simulink library "Linkage_Shock"  (R2025a)
settings: Solver=VariableStepAuto  StartTime=0.0  StopTime=10.0  RelTol=1e-3
undefined symbols (not defined in the file): bumpstop_len_shock, clr_conn_shock, clr_shock_bumpstop, clr_shock_cyl, clr_shock_piston, cyl_cap_len_shock, deadvol_len_shock_cyl, hp_spr_bot, hp_spr_top, low_lim_bumpstop, opc_conn_shock, opc_shock_bumpstop, opc_shock_cyl, opc_shock_piston, piston_len_shock, radius_shock_cyl, shock_cyl_mass, shock_pist_mass, size_conn_shock, up_lim_bumpstop, Vehicle, Visual, X, Y, Z
libraries: sm_lib x36, nesl_utility x9, fl_lib x3, Suspension_Utilities x3
(part 1 of 2)
Description:
  | Component of Simscape Vehicle Templates Library
  | 
  | Copyright 2018-2026 The MathWorks, Inc.
settings Model: Creator=smiller  LastModifiedBy=smiller
settings SolverCC: AlgebraicLoopSolver=TrustRegion
settings DataIOCC: ReturnWorkspaceOutputs=off
settings OptimizationCC: ReuseModelBlockBuffer=off
settings DebuggingCC: UnconnectedInputMsg=warning  UnconnectedOutputMsg=warning  UnconnectedLineMsg=warning  ArithmeticOperatorsInVariantConditions=warning
settings ModelReferenceCC: EnableRefExpFcnMdlSchedulingChecks=on
settings SFSimCC: CustomCodeUndefinedFunction=UseInterfaceOnly
settings RTWCC: GPUComputeCapability=3.5

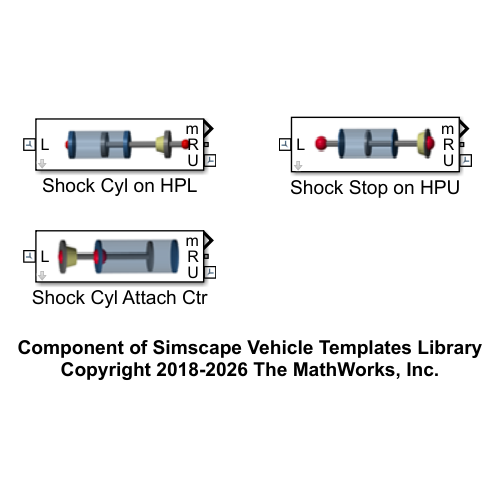
[thumbnail: Simulink's stored preview of the top-level diagram]
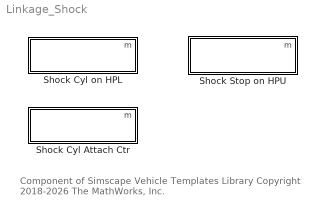
== system Linkage_Shock ==
  note: Component of Simscape Vehicle Templates Library
      | Copyright 2018-2026 The MathWorks, Inc.
  Shock Cyl Attach Ctr : Subsystem  mask(Shock Absorber Parts){shock_pist_mass=Vehicle.Chassis.SuspA1.AxleTA2PR.Shock.mPiston.Value, shock_cyl_mass=Vehicle.Chassis.SuspA1.AxleTA2PR.Shock.mCylinder.Value, hp_spr_top=Vehicle.Chassis.SuspA1.AxleTA2PR.Shock.sTop.Value, hp_spr_bot=Vehicle.Chassis.SuspA1.AxleTA2PR.Shock.sBottom.Value, up_lim_bumpstop=Vehicle.Chassis.SuspA1.AxleTA2PR.Endstop.xMax.Value, low_lim_bumpstop=Vehicle.Chassis.SuspA1.AxleTA2PR.Endstop.xMin.Value, clr_conn_shock=Visual.hp.clr, opc_conn_shock=Visual.hp.opc, size_conn_shock=Visual.hp.rad, clr_shock_cyl=Visual.clr.blue, opc_shock_cyl=Visual.part.opc, radius_shock_cyl=0.05, clr_shock_piston=Visual.clr.gray, opc_shock_piston=Visual.part.opc, clr_shock_bumpstop=Visual.clr.yellowpale, opc_shock_bumpstop=Visual.part.opc, deadvol_len_shock_cyl=Visual.Shock.dead_length, piston_len_shock=Visual.Shock.piston.len, cyl_cap_len_shock=Visual.Shock.cap.len, bumpstop_len_shock=Visual.Shock.bumpstop.len}
      mask prompts: shock_pist_mass "Piston Mass (kg)"; shock_cyl_mass "Cylinder Mass (kg)"; hp_spr_top "Spring Top [xyz] (m)"; hp_spr_bot "Spring Bottom [xyz] (m)"; up_lim_bumpstop "Upper Limit Bumpstop (m)"; low_lim_bumpstop "Lower Limit Bumpstop (m)"; deadvol_len_shock_cyl "Dead Volume Height (m)"; piston_len_shock "Piston Length (m)"; cyl_cap_len_shock "Cylinder Cap Length (m)"; bumpstop_len_shock "Bumpstop Length (m)"
      mask help: Models mechanical parts of shock absorber.
      mask init:
      | init_spr_len = norm(hp_spr_top-hp_spr_bot);
      | 
      | rod_length = init_spr_len+abs(up_lim_bumpstop)+piston_len_shock;
      | 
      | bumpstop_xc_rev = [0 0; 0.5 0; 0.7 1; 0 1].*[radius_shock_cyl bumpstop_len_shock];
      | 
      | cyl_wall_length = piston_len_shock+abs(low_lim_bumpstop)+abs(up_lim_bumpstop)+deadvol_len_shock_cyl;
      mask Help: web('sm_car_doc_susp_shock.html')
      mask TypeOptions shock_pist_mass: Piston/Rod/Mass
      mask TypeOptions shock_cyl_mass: Cylinder/Wall/Mass
      mask TypeOptions clr_conn_shock:
      | Vis
      | Spring
      | LA/GraphicDiffuseColor | Vis
      | Spring
      | HP/GraphicDiffuseColor
      mask TypeOptions opc_conn_shock:
      | Vis
      | Spring
      | LA/GraphicOpacity | Vis
      | Spring
      | HP/GraphicOpacity
      mask TypeOptions clr_shock_cyl: Cylinder/Cap Bottom/GraphicDiffuseColor | Cylinder/Cap Top/GraphicDiffuseColor | Cylinder/Wall/GraphicDiffuseColor
      mask TypeOptions clr_shock_piston: Piston/Cap/GraphicDiffuseColor | Piston/Piston/GraphicDiffuseColor | Piston/Rod/GraphicDiffuseColor
      mask TypeOptions opc_shock_piston: Piston/Cap/GraphicOpacity | Piston/Piston/GraphicOpacity | Piston/Rod/GraphicOpacity
      mask TypeOptions clr_shock_bumpstop: Piston/Bumpstop/GraphicDiffuseColor
      mask TypeOptions opc_shock_bumpstop: Piston/Bumpstop/GraphicOpacity
      mask DialogControl cont_shock Prompt: Shock
      mask DialogControl cont_vis_shock Prompt: Visualization
      mask DialogControl text_clr_shock Prompt: Color  [RGB]
      mask DialogControl text_opc_shock Prompt: Opac. (0-1)
      mask DialogControl text_size_shock Prompt: Size (m)
      mask DialogControl text_conn_shock Prompt: Connections
      mask DialogControl text_shock_cyl Prompt: Cylinder
      mask DialogControl text_shock_piston Prompt: Piston
      mask DialogControl text_piston_radius Prompt: <cylinder radius>
      mask DialogControl text_shock_bumpstop Prompt: Bumpstop
      mask DialogControl text_bumpstop_radius Prompt: <cylinder radius>
      mask Display: image('sm_car_vehicle_linkage_shock_hpc_IMAGE.png');
  Shock Cyl on HPL : Subsystem  mask{shock_pist_mass=shock_pist_mass, shock_cyl_mass=shock_cyl_mass, hp_spr_top=hp_spr_top, hp_spr_bot=hp_spr_bot, up_lim_bumpstop=up_lim_bumpstop, low_lim_bumpstop=low_lim_bumpstop, clr_conn_shock=clr_conn_shock, opc_conn_shock=opc_conn_shock, size_conn_shock=size_conn_shock, clr_shock_cyl=clr_shock_cyl, opc_shock_cyl=opc_shock_cyl, radius_shock_cyl=radius_shock_cyl, clr_shock_piston=clr_shock_piston, opc_shock_piston=opc_shock_piston, clr_shock_bumpstop=clr_shock_bumpstop, opc_shock_bumpstop=opc_shock_bumpstop, deadvol_len_shock_cyl=deadvol_len_shock_cyl, piston_len_shock=piston_len_shock, cyl_cap_len_shock=cyl_cap_len_shock, bumpstop_len_shock=bumpstop_len_shock}
      mask prompts: shock_pist_mass "Piston Mass (kg)"; shock_cyl_mass "Cylinder Mass (kg)"; hp_spr_top "Shock Top [xyz] (m)"; hp_spr_bot "Shock Bottom [xyz] (m)"; up_lim_bumpstop "Upper Limit Bumpstop (m)"; low_lim_bumpstop "Lower Limit Bumpstop (m)"; deadvol_len_shock_cyl "Dead Volume Height (m)"; piston_len_shock "Piston Length (m)"; cyl_cap_len_shock "Cylinder Cap Length (m)"; bumpstop_len_shock "Bumpstop Length (m)"
      mask init:
      | init_spr_len = norm(hp_spr_top-hp_spr_bot);
      | 
      | rod_length = init_spr_len-deadvol_len_shock_cyl-cyl_cap_len_shock-abs(low_lim_bumpstop);
      | 
      | bumpstop_xc_rev = [0 0; 0.7 0; 0.9 1; 0 1].*[radius_shock_cyl bumpstop_len_shock];
      | 
      | cyl_wall_length = piston_len_shock+abs(low_lim_bumpstop)+abs(up_lim_bumpstop)+deadvol_len_shock_cyl;
      mask Help: web('sm_car_doc_susp_shock.html')
      mask TypeOptions shock_pist_mass: Piston/Rod/Mass
      mask TypeOptions shock_cyl_mass: Cylinder/Wall/Mass
      mask TypeOptions clr_conn_shock:
      | Vis
      | HP L/GraphicDiffuseColor | Vis
      | HP U/GraphicDiffuseColor
      mask TypeOptions opc_conn_shock:
      | Vis
      | HP L/GraphicOpacity | Vis
      | HP U/GraphicOpacity
      mask TypeOptions clr_shock_cyl: Cylinder/Cap Bottom/GraphicDiffuseColor | Cylinder/Cap Top/GraphicDiffuseColor | Cylinder/Wall/GraphicDiffuseColor
      mask TypeOptions clr_shock_piston: Piston/Cap/GraphicDiffuseColor | Piston/Piston/GraphicDiffuseColor | Piston/Rod/GraphicDiffuseColor
      mask TypeOptions opc_shock_piston: Piston/Cap/GraphicOpacity | Piston/Piston/GraphicOpacity | Piston/Rod/GraphicOpacity
      mask TypeOptions clr_shock_bumpstop: Piston/Bumpstop/GraphicDiffuseColor
      mask TypeOptions opc_shock_bumpstop: Piston/Bumpstop/GraphicOpacity
      mask DialogControl cont_shock Prompt: Shock
      mask DialogControl cont_vis_shock Prompt: Visualization
      mask DialogControl text_blank_shock Prompt: (Add text here)
      mask DialogControl text_clr_shock Prompt: Color  [RGB]
      mask DialogControl text_opc_shock Prompt: Opac. (0-1)
      mask DialogControl text_size_shock Prompt: Size (m)
      mask DialogControl text_conn_shock Prompt: Connections
      mask DialogControl text_shock_cyl Prompt: Cylinder
      mask DialogControl text_shock_piston Prompt: Piston
      mask DialogControl text_piston_radius Prompt: <cylinder radius>
      mask DialogControl text_shock_bumpstop Prompt: Bumpstop
      mask DialogControl text_bumpstop_radius Prompt: <cylinder radius>
      mask Display: image('sm_car_vehicle_linkage_shock_IMAGE.png');
  Shock Stop on HPU : Subsystem  mask{shock_pist_mass=shock_pist_mass, shock_cyl_mass=shock_cyl_mass, hp_spr_top=hp_spr_top, hp_spr_bot=hp_spr_bot, up_lim_bumpstop=up_lim_bumpstop, low_lim_bumpstop=low_lim_bumpstop, clr_conn_shock=clr_conn_shock, opc_conn_shock=opc_conn_shock, size_conn_shock=size_conn_shock, clr_shock_cyl=clr_shock_cyl, opc_shock_cyl=opc_shock_cyl, radius_shock_cyl=radius_shock_cyl, clr_shock_piston=clr_shock_piston, opc_shock_piston=opc_shock_piston, clr_shock_bumpstop=clr_shock_bumpstop, opc_shock_bumpstop=opc_shock_bumpstop, deadvol_len_shock_cyl=deadvol_len_shock_cyl, piston_len_shock=piston_len_shock, cyl_cap_len_shock=cyl_cap_len_shock, bumpstop_len_shock=bumpstop_len_shock}
      mask prompts: shock_pist_mass "Piston Mass (kg)"; shock_cyl_mass "Cylinder Mass (kg)"; hp_spr_top "Shock Top [xyz] (m)"; hp_spr_bot "Shock Bottom [xyz] (m)"; up_lim_bumpstop "Upper Limit Bumpstop (m)"; low_lim_bumpstop "Lower Limit Bumpstop (m)"; deadvol_len_shock_cyl "Dead Volume Height (m)"; piston_len_shock "Piston Length (m)"; cyl_cap_len_shock "Cylinder Cap Length (m)"; bumpstop_len_shock "Bumpstop Length (m)"
      mask init:
      | init_spr_len = norm(hp_spr_top-hp_spr_bot);
      | 
      | rod_length_upper = ...
      | cyl_cap_len_shock + bumpstop_len_shock + abs(low_lim_bumpstop) + ...
      | cyl_cap_len_shock + abs(up_lim_bumpstop) + piston_len_shock;
      | 
      | rod_length_lower = init_spr_len - rod_length_upper - deadvol_len_shock_cyl - cyl_cap_len_shock - abs(low_lim_bumpstop);
      | 
      | bumpstop_xc_rev = [0 0; 0.7 0; 0.9 1; 0 1].*[radius_shock_cyl bumpstop_len_shock];
      | 
      | cyl_wall_length = piston_len_shock+abs(low_lim_bumpstop)+abs(up_lim_bumpstop)+deadvol_len_shock_cyl;
      mask Help: web('sm_car_doc_susp_shock.html')
      mask TypeOptions shock_pist_mass: Piston/Rod/Mass
      mask TypeOptions shock_cyl_mass: Cylinder/Wall/Mass
      mask TypeOptions clr_conn_shock:
      | Vis
      | HP L/GraphicDiffuseColor | Vis
      | HP U/GraphicDiffuseColor
      mask TypeOptions opc_conn_shock:
      | Vis
      | HP L/GraphicOpacity | Vis
      | HP U/GraphicOpacity
      mask TypeOptions clr_shock_cyl: Cylinder/Cap Bottom/GraphicDiffuseColor | Cylinder/Cap Top/GraphicDiffuseColor | Cylinder/Wall/GraphicDiffuseColor
      mask TypeOptions clr_shock_piston: Piston/Cap/GraphicDiffuseColor | Piston/Piston/GraphicDiffuseColor | Piston/Rod/GraphicDiffuseColor
      mask TypeOptions opc_shock_piston: Piston/Cap/GraphicOpacity | Piston/Piston/GraphicOpacity | Piston/Rod/GraphicOpacity
      mask TypeOptions clr_shock_bumpstop: Piston/Bumpstop/GraphicDiffuseColor
      mask TypeOptions opc_shock_bumpstop: Piston/Bumpstop/GraphicOpacity
      mask DialogControl cont_shock Prompt: Shock
      mask DialogControl cont_vis_shock Prompt: Visualization
      mask DialogControl text_blank_shock Prompt: (Add text here)
      mask DialogControl text_clr_shock Prompt: Color  [RGB]
      mask DialogControl text_opc_shock Prompt: Opac. (0-1)
      mask DialogControl text_size_shock Prompt: Size (m)
      mask DialogControl text_conn_shock Prompt: Connections
      mask DialogControl text_shock_cyl Prompt: Cylinder
      mask DialogControl text_shock_piston Prompt: Piston
      mask DialogControl text_piston_radius Prompt: <cylinder radius>
      mask DialogControl text_shock_bumpstop Prompt: Bumpstop
      mask DialogControl text_bumpstop_radius Prompt: <cylinder radius>
      mask Display: image('sm_car_vehicle_linkage_shock_hpu_IMAGE.png');

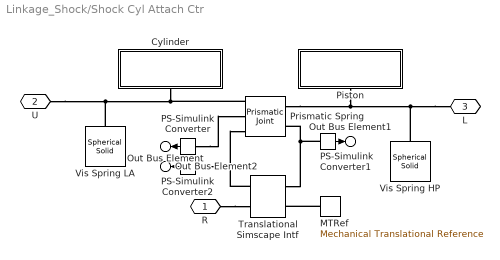
== system Linkage_Shock/Shock Cyl Attach Ctr ==
  Cylinder : Subsystem
  MTRef : fl_lib/Mechanical/Translational Elements/Mechanical Translational Reference
  PS-Simulink Converter : nesl_utility/PS-Simulink Converter  PhysicalDomain=network_engine_domain  SubClassName=ps_output  LeftPortType=input  RightPortType=output  PseudoPeriodic=off  Frequencies=[]  VectorFormat=1-D array  Unit=1  AffineConversion=off
  PS-Simulink Converter1 : nesl_utility/PS-Simulink Converter  PhysicalDomain=network_engine_domain  SubClassName=ps_output  LeftPortType=input  RightPortType=output  PseudoPeriodic=off  Frequencies=[]  VectorFormat=1-D array  Unit=1  AffineConversion=off
  PS-Simulink Converter2 : nesl_utility/PS-Simulink Converter  PhysicalDomain=network_engine_domain  SubClassName=ps_output  LeftPortType=input  RightPortType=output  PseudoPeriodic=off  Frequencies=[]  VectorFormat=1-D array  Unit=1  AffineConversion=off
  Piston : Subsystem
  Prismatic Spring : sm_lib/Joints/Prismatic Joint  JointMode=Normal  CompositeWrenchDir=FollowerOnBase  CompositeWrenchFrame=BaseFrame  SenseConstraintForce=off  SenseConstraintTorque=off  SenseTotalForce=off  SenseTotalTorque=off  PositionTargetSpecify=on  PositionTargetPriority=Low  PositionTargetValue=init_spr_len  PositionTargetValueUnits=m  VelocityTargetSpecify=off  VelocityTargetPriority=High  VelocityTargetValue=0  VelocityTargetValueUnits=m/s  EquilibriumPosition=0  EquilibriumPositionUnits=m  SpringStiffness=0  SpringStiffnessUnits=N/m  DampingCoefficient=0.01  DampingCoefficientUnits=N/(m/s)  LowerLimitSpecify=off  LowerLimitBound=-1  LowerLimitBoundUnits=m  LowerLimitStiffness=1e6  LowerLimitStiffnessUnits=N/m  LowerLimitDamping=1e3  LowerLimitDampingUnits=N/(m/s)  LowerLimitTransitionRegionWidth=1e-4  LowerLimitTransitionRegionWidthUnits=m  UpperLimitSpecify=off  UpperLimitBound=1  UpperLimitBoundUnits=m  UpperLimitStiffness=1e6  UpperLimitStiffnessUnits=N/m  UpperLimitDamping=1e3  UpperLimitDampingUnits=N/(m/s)  UpperLimitTransitionRegionWidth=1e-4  UpperLimitTransitionRegionWidthUnits=m  TorqueActuationMode=InputTorque  MotionActuationMode=ComputedMotion  SensePosition=on  SenseVelocity=on  SenseAcceleration=off  SenseTorqueForce=off  SenseLowerLimitTorqueForce=off  SenseUpperLimitTorqueForce=off
  Translational Simscape Intf : Suspension_Utilities/Translational Simscape Intf  SystemSampleTime=-1  VariantActivationTime=update diagram  EmptyChoice=off  PassThrough=off  PassThroughVariantControl=(default)  EmptyChoiceVariantControl=(default)  AllowFlexibleInterface=on  Latency=0  AutoFrameSizeCalculation=off
  Vis Spring HP : sm_lib/Body Elements/Spherical Solid  SphereRadius=size_conn_shock  SphereRadiusUnits=m  ExportEntireGeometry=off  InertiaType=PointMass  BasedOnType=Density  Density=0  DensityUnits=kg/m^3  Mass=0  MassUnits=kg  CenterOfMass=[0 0 0]  CenterOfMassUnits=m  MomentsOfInertia=[1 1 1]  MomentsOfInertiaUnits=kg*m^2  ProductsOfInertia=[0 0 0]  ProductsOfInertiaUnits=kg*m^2  GraphicType=FromGeometry  MarkerShape=Sphere  MarkerSize=10  GraphicVisPropType=SimpleVisualProperties  GraphicDiffuseColor=clr_conn_shock  GraphicOpacity=opc_conn_shock  GraphicSpecularColor=[0.5 0.5 0.5 1.0]  GraphicAmbientColor=[0.15 0.15 0.15 1.0]  GraphicEmissiveColor=[0.0 0.0 0.0 1.0]  GraphicShininess=75  DoExposeReferenceFrame=on  SerializedFrames=<Frames/>
  Vis Spring LA : sm_lib/Body Elements/Spherical Solid  SphereRadius=size_conn_shock  SphereRadiusUnits=m  ExportEntireGeometry=off  InertiaType=PointMass  BasedOnType=Density  Density=0  DensityUnits=kg/m^3  Mass=0  MassUnits=kg  CenterOfMass=[0 0 0]  CenterOfMassUnits=m  MomentsOfInertia=[1 1 1]  MomentsOfInertiaUnits=kg*m^2  ProductsOfInertia=[0 0 0]  ProductsOfInertiaUnits=kg*m^2  GraphicType=FromGeometry  MarkerShape=Sphere  MarkerSize=10  GraphicVisPropType=SimpleVisualProperties  GraphicDiffuseColor=clr_conn_shock  GraphicOpacity=opc_conn_shock  GraphicSpecularColor=[0.5 0.5 0.5 1.0]  GraphicAmbientColor=[0.15 0.15 0.15 1.0]  GraphicEmissiveColor=[0.0 0.0 0.0 1.0]  GraphicShininess=75  DoExposeReferenceFrame=on  SerializedFrames=<Frames/>
  R : PMIOPort  Side=Right
  U : PMIOPort  Port=2  Side=Right
  L : PMIOPort  Port=3  Side=Left
  Out Bus Element : Outport  VectorParamsAs1DForOutWhenUnconnected=off  PortName=m  Element=x
  Out Bus Element1 : Outport  VectorParamsAs1DForOutWhenUnconnected=off  PortName=m  Element=f
  Out Bus Element2 : Outport  VectorParamsAs1DForOutWhenUnconnected=off  PortName=m  Element=v
  wires:
  PS-Simulink Converter/1 -> Out Bus Element/1
  PS-Simulink Converter1/1 -> Out Bus Element1/1
  PS-Simulink Converter2/1 -> Out Bus Element2/1
  connections:
  R/RConn1 -- Translational Simscape Intf/RConn2
  MTRef/LConn1 -- Translational Simscape Intf/LConn2
  L/RConn1 -- Prismatic Spring/LConn1 -- Piston/RConn1 -- Vis Spring HP/RConn1
  Cylinder/LConn1 -- U/RConn1 -- Vis Spring LA/RConn1 -- Prismatic Spring/RConn1
  Translational Simscape Intf/RConn1 -- PS-Simulink Converter2/LConn1 -- Prismatic Spring/RConn3
  Translational Simscape Intf/LConn1 -- PS-Simulink Converter1/LConn1 -- Prismatic Spring/LConn2
  PS-Simulink Converter/LConn1 -- Prismatic Spring/RConn2

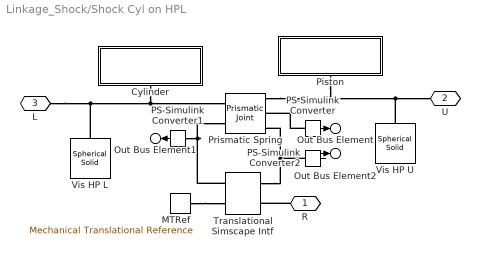
== system Linkage_Shock/Shock Cyl on HPL ==
  Cylinder : Subsystem
  MTRef : fl_lib/Mechanical/Translational Elements/Mechanical Translational Reference
  PS-Simulink Converter : nesl_utility/PS-Simulink Converter  PhysicalDomain=network_engine_domain  SubClassName=ps_output  LeftPortType=input  RightPortType=output  PseudoPeriodic=off  Frequencies=[]  VectorFormat=1-D array  Unit=m  AffineConversion=off
  PS-Simulink Converter1 : nesl_utility/PS-Simulink Converter  PhysicalDomain=network_engine_domain  SubClassName=ps_output  LeftPortType=input  RightPortType=output  PseudoPeriodic=off  Frequencies=[]  VectorFormat=1-D array  Unit=N  AffineConversion=off
  PS-Simulink Converter2 : nesl_utility/PS-Simulink Converter  PhysicalDomain=network_engine_domain  SubClassName=ps_output  LeftPortType=input  RightPortType=output  PseudoPeriodic=off  Frequencies=[]  VectorFormat=1-D array  Unit=m/s  AffineConversion=off
  Piston : Subsystem
  Prismatic Spring : sm_lib/Joints/Prismatic Joint  JointMode=Normal  CompositeWrenchDir=FollowerOnBase  CompositeWrenchFrame=BaseFrame  SenseConstraintForce=off  SenseConstraintTorque=off  SenseTotalForce=off  SenseTotalTorque=off  PositionTargetSpecify=on  PositionTargetPriority=High  PositionTargetValue=init_spr_len  PositionTargetValueUnits=m  VelocityTargetSpecify=off  VelocityTargetPriority=High  VelocityTargetValue=0  VelocityTargetValueUnits=m/s  EquilibriumPosition=0  EquilibriumPositionUnits=m  SpringStiffness=0  SpringStiffnessUnits=N/m  DampingCoefficient=0.01  DampingCoefficientUnits=N/(m/s)  LowerLimitSpecify=off  LowerLimitBound=-1  LowerLimitBoundUnits=m  LowerLimitStiffness=1e6  LowerLimitStiffnessUnits=N/m  LowerLimitDamping=1e3  LowerLimitDampingUnits=N/(m/s)  LowerLimitTransitionRegionWidth=1e-4  LowerLimitTransitionRegionWidthUnits=m  UpperLimitSpecify=off  UpperLimitBound=1  UpperLimitBoundUnits=m  UpperLimitStiffness=1e6  UpperLimitStiffnessUnits=N/m  UpperLimitDamping=1e3  UpperLimitDampingUnits=N/(m/s)  UpperLimitTransitionRegionWidth=1e-4  UpperLimitTransitionRegionWidthUnits=m  TorqueActuationMode=InputTorque  MotionActuationMode=ComputedMotion  SensePosition=on  SenseVelocity=on  SenseAcceleration=off  SenseTorqueForce=off  SenseLowerLimitTorqueForce=off  SenseUpperLimitTorqueForce=off
  Translational Simscape Intf : Suspension_Utilities/Translational Simscape Intf  SystemSampleTime=-1  VariantActivationTime=update diagram  EmptyChoice=off  PassThrough=off  PassThroughVariantControl=(default)  EmptyChoiceVariantControl=(default)  AllowFlexibleInterface=on  Latency=0  AutoFrameSizeCalculation=off
  Vis HP L : sm_lib/Body Elements/Spherical Solid  SphereRadius=size_conn_shock  SphereRadiusUnits=m  ExportEntireGeometry=off  InertiaType=PointMass  BasedOnType=Density  Density=0  DensityUnits=kg/m^3  Mass=0  MassUnits=kg  CenterOfMass=[0 0 0]  CenterOfMassUnits=m  MomentsOfInertia=[1 1 1]  MomentsOfInertiaUnits=kg*m^2  ProductsOfInertia=[0 0 0]  ProductsOfInertiaUnits=kg*m^2  GraphicType=FromGeometry  MarkerShape=Sphere  MarkerSize=10  GraphicVisPropType=SimpleVisualProperties  GraphicDiffuseColor=clr_conn_shock  GraphicOpacity=opc_conn_shock  GraphicSpecularColor=[0.5 0.5 0.5 1.0]  GraphicAmbientColor=[0.15 0.15 0.15 1.0]  GraphicEmissiveColor=[0.0 0.0 0.0 1.0]  GraphicShininess=75  DoExposeReferenceFrame=on  SerializedFrames=<Frames/>
  Vis HP U : sm_lib/Body Elements/Spherical Solid  SphereRadius=size_conn_shock  SphereRadiusUnits=m  ExportEntireGeometry=off  InertiaType=PointMass  BasedOnType=Density  Density=0  DensityUnits=kg/m^3  Mass=0  MassUnits=kg  CenterOfMass=[0 0 0]  CenterOfMassUnits=m  MomentsOfInertia=[1 1 1]  MomentsOfInertiaUnits=kg*m^2  ProductsOfInertia=[0 0 0]  ProductsOfInertiaUnits=kg*m^2  GraphicType=FromGeometry  MarkerShape=Sphere  MarkerSize=10  GraphicVisPropType=SimpleVisualProperties  GraphicDiffuseColor=clr_conn_shock  GraphicOpacity=opc_conn_shock  GraphicSpecularColor=[0.5 0.5 0.5 1.0]  GraphicAmbientColor=[0.15 0.15 0.15 1.0]  GraphicEmissiveColor=[0.0 0.0 0.0 1.0]  GraphicShininess=75  DoExposeReferenceFrame=on  SerializedFrames=<Frames/>
  R : PMIOPort  Side=Right
  U : PMIOPort  Port=2  Side=Right
  L : PMIOPort  Port=3  Side=Left
  Out Bus Element : Outport  VectorParamsAs1DForOutWhenUnconnected=off  PortName=m  Element=x
  Out Bus Element1 : Outport  VectorParamsAs1DForOutWhenUnconnected=off  PortName=m  Element=f
  Out Bus Element2 : Outport  VectorParamsAs1DForOutWhenUnconnected=off  PortName=m  Element=v
  wires:
  PS-Simulink Converter/1 -> Out Bus Element/1
  PS-Simulink Converter1/1 -> Out Bus Element1/1
  PS-Simulink Converter2/1 -> Out Bus Element2/1
  connections:
  Translational Simscape Intf/LConn1 -- PS-Simulink Converter1/LConn1 -- Prismatic Spring/LConn2
  Translational Simscape Intf/RConn1 -- PS-Simulink Converter2/LConn1 -- Prismatic Spring/RConn3
  Vis HP L/RConn1 -- Cylinder/LConn1 -- Prismatic Spring/LConn1 -- L/RConn1
  Vis HP U/RConn1 -- Piston/RConn1 -- Prismatic Spring/RConn1 -- U/RConn1
  MTRef/LConn1 -- Translational Simscape Intf/LConn2
  R/RConn1 -- Translational Simscape Intf/RConn2
  PS-Simulink Converter/LConn1 -- Prismatic Spring/RConn2

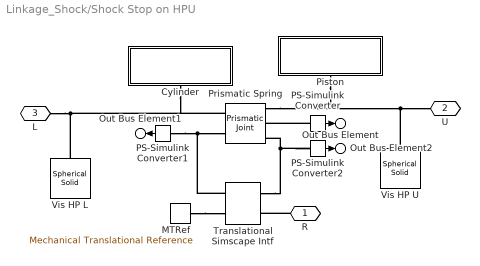
== system Linkage_Shock/Shock Stop on HPU ==
  Cylinder : Subsystem
  MTRef : fl_lib/Mechanical/Translational Elements/Mechanical Translational Reference
  PS-Simulink Converter : nesl_utility/PS-Simulink Converter  PhysicalDomain=network_engine_domain  SubClassName=ps_output  LeftPortType=input  RightPortType=output  PseudoPeriodic=off  Frequencies=[]  VectorFormat=1-D array  Unit=m  AffineConversion=off
  PS-Simulink Converter1 : nesl_utility/PS-Simulink Converter  PhysicalDomain=network_engine_domain  SubClassName=ps_output  LeftPortType=input  RightPortType=output  PseudoPeriodic=off  Frequencies=[]  VectorFormat=1-D array  Unit=N  AffineConversion=off
  PS-Simulink Converter2 : nesl_utility/PS-Simulink Converter  PhysicalDomain=network_engine_domain  SubClassName=ps_output  LeftPortType=input  RightPortType=output  PseudoPeriodic=off  Frequencies=[]  VectorFormat=1-D array  Unit=m/s  AffineConversion=off
  Piston : Subsystem
  Prismatic Spring : sm_lib/Joints/Prismatic Joint  JointMode=Normal  CompositeWrenchDir=FollowerOnBase  CompositeWrenchFrame=BaseFrame  SenseConstraintForce=off  SenseConstraintTorque=off  SenseTotalForce=off  SenseTotalTorque=off  PositionTargetSpecify=on  PositionTargetPriority=High  PositionTargetValue=init_spr_len  PositionTargetValueUnits=m  VelocityTargetSpecify=off  VelocityTargetPriority=High  VelocityTargetValue=0  VelocityTargetValueUnits=m/s  EquilibriumPosition=0  EquilibriumPositionUnits=m  SpringStiffness=0  SpringStiffnessUnits=N/m  DampingCoefficient=0  DampingCoefficientUnits=N/(m/s)  LowerLimitSpecify=off  LowerLimitBound=-1  LowerLimitBoundUnits=m  LowerLimitStiffness=1e6  LowerLimitStiffnessUnits=N/m  LowerLimitDamping=1e3  LowerLimitDampingUnits=N/(m/s)  LowerLimitTransitionRegionWidth=1e-4  LowerLimitTransitionRegionWidthUnits=m  UpperLimitSpecify=off  UpperLimitBound=1  UpperLimitBoundUnits=m  UpperLimitStiffness=1e6  UpperLimitStiffnessUnits=N/m  UpperLimitDamping=1e3  UpperLimitDampingUnits=N/(m/s)  UpperLimitTransitionRegionWidth=1e-4  UpperLimitTransitionRegionWidthUnits=m  TorqueActuationMode=InputTorque  MotionActuationMode=ComputedMotion  SensePosition=on  SenseVelocity=on  SenseAcceleration=off  SenseTorqueForce=off  SenseLowerLimitTorqueForce=off  SenseUpperLimitTorqueForce=off
  Translational Simscape Intf : Suspension_Utilities/Translational Simscape Intf  SystemSampleTime=-1  VariantActivationTime=update diagram  EmptyChoice=off  PassThrough=off  PassThroughVariantControl=(default)  EmptyChoiceVariantControl=(default)  AllowFlexibleInterface=on  Latency=0  AutoFrameSizeCalculation=off
  Vis HP L : sm_lib/Body Elements/Spherical Solid  SphereRadius=size_conn_shock  SphereRadiusUnits=m  ExportEntireGeometry=off  InertiaType=PointMass  BasedOnType=Density  Density=0  DensityUnits=kg/m^3  Mass=0  MassUnits=kg  CenterOfMass=[0 0 0]  CenterOfMassUnits=m  MomentsOfInertia=[1 1 1]  MomentsOfInertiaUnits=kg*m^2  ProductsOfInertia=[0 0 0]  ProductsOfInertiaUnits=kg*m^2  GraphicType=FromGeometry  MarkerShape=Sphere  MarkerSize=10  GraphicVisPropType=SimpleVisualProperties  GraphicDiffuseColor=clr_conn_shock  GraphicOpacity=opc_conn_shock  GraphicSpecularColor=[0.5 0.5 0.5 1.0]  GraphicAmbientColor=[0.15 0.15 0.15 1.0]  GraphicEmissiveColor=[0.0 0.0 0.0 1.0]  GraphicShininess=75  DoExposeReferenceFrame=on  SerializedFrames=<Frames/>
  Vis HP U : sm_lib/Body Elements/Spherical Solid  SphereRadius=size_conn_shock  SphereRadiusUnits=m  ExportEntireGeometry=off  InertiaType=PointMass  BasedOnType=Density  Density=0  DensityUnits=kg/m^3  Mass=0  MassUnits=kg  CenterOfMass=[0 0 0]  CenterOfMassUnits=m  MomentsOfInertia=[1 1 1]  MomentsOfInertiaUnits=kg*m^2  ProductsOfInertia=[0 0 0]  ProductsOfInertiaUnits=kg*m^2  GraphicType=FromGeometry  MarkerShape=Sphere  MarkerSize=10  GraphicVisPropType=SimpleVisualProperties  GraphicDiffuseColor=clr_conn_shock  GraphicOpacity=opc_conn_shock  GraphicSpecularColor=[0.5 0.5 0.5 1.0]  GraphicAmbientColor=[0.15 0.15 0.15 1.0]  GraphicEmissiveColor=[0.0 0.0 0.0 1.0]  GraphicShininess=75  DoExposeReferenceFrame=on  SerializedFrames=<Frames/>
  R : PMIOPort  Side=Right
  U : PMIOPort  Port=2  Side=Right
  L : PMIOPort  Port=3  Side=Left
  Out Bus Element : Outport  VectorParamsAs1DForOutWhenUnconnected=off  PortName=m  Element=x
  Out Bus Element1 : Outport  VectorParamsAs1DForOutWhenUnconnected=off  PortName=m  Element=f
  Out Bus Element2 : Outport  VectorParamsAs1DForOutWhenUnconnected=off  PortName=m  Element=v
  wires:
  PS-Simulink Converter/1 -> Out Bus Element/1
  PS-Simulink Converter1/1 -> Out Bus Element1/1
  PS-Simulink Converter2/1 -> Out Bus Element2/1
  connections:
  R/RConn1 -- Translational Simscape Intf/RConn2
  MTRef/LConn1 -- Translational Simscape Intf/LConn2
  Piston/RConn1 -- Prismatic Spring/RConn1 -- Vis HP U/RConn1 -- U/RConn1
  Translational Simscape Intf/RConn1 -- PS-Simulink Converter2/LConn1 -- Prismatic Spring/RConn3
  Translational Simscape Intf/LConn1 -- PS-Simulink Converter1/LConn1 -- Prismatic Spring/LConn2
  L/RConn1 -- Prismatic Spring/LConn1 -- Cylinder/LConn1 -- Vis HP L/RConn1
  PS-Simulink Converter/LConn1 -- Prismatic Spring/RConn2

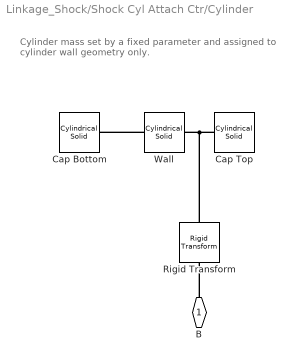
== system Linkage_Shock/Shock Cyl Attach Ctr/Cylinder ==
  note: Cylinder mass set by a fixed parameter
      | and assigned to cylinder wall geometry only.
  Cap Bottom : sm_lib/Body Elements/Cylindrical Solid  CylinderRadius=radius_shock_cyl  CylinderRadiusUnits=m  CylinderLength=cyl_cap_len_shock  CylinderLengthUnits=m  ExportEntireGeometry=off  InertiaType=CalculateFromGeometry  BasedOnType=Density  Density=0  DensityUnits=kg/m^3  Mass=1  MassUnits=kg  CenterOfMass=[0 0 0]  CenterOfMassUnits=m  MomentsOfInertia=[1 1 1]  MomentsOfInertiaUnits=kg*m^2  ProductsOfInertia=[0 0 0]  ProductsOfInertiaUnits=kg*m^2  GraphicType=FromGeometry  MarkerShape=Sphere  MarkerSize=10  GraphicVisPropType=SimpleVisualProperties  GraphicDiffuseColor=clr_shock_cyl  GraphicOpacity=opc_shock_cyl  GraphicSpecularColor=[0.5 0.5 0.5 1.0]  GraphicAmbientColor=[0.15 0.15 0.15 1.0]  GraphicEmissiveColor=[0.0 0.0 0.0 1.0]  GraphicShininess=75  DoExposeReferenceFrame=off  SerializedFrames=<Frames><Frame><Id>Frame1</Id><Value><Name>F</Name><Origin><Source>GeometricFeature</Source><FeatureName>top surface</FeatureName></Origin><PrimaryAxis><DefinedDirection>+Z</DefinedDirection><Source>ReferenceFrame</Source><SourceDirection>+Z</SourceDirection><FeatureName></FeatureName></PrimaryAxis><SecondaryAxis><DefinedDirection>+X</DefinedDirection><Source>ReferenceFrame</Source><SourceDirection>+X</SourceDirection><FeatureName></FeatureName></SecondaryAxis></Value></Frame><Frame><Id>Frame2</Id><Value><Name>B</Name><Origin><Source>GeometricFeature</Source><FeatureName>bottom surface</FeatureName></Origin><PrimaryAxis><DefinedDirection>+Z</DefinedDirection><Source>ReferenceFrame</Source><SourceDirection>+Z</SourceDirection><FeatureName></FeatureName></PrimaryAxis><SecondaryAxis><DefinedDirection>+X</DefinedDirection><Source>ReferenceFrame</Source><SourceDirection>+X</SourceDirection><FeatureName></FeatureName></SecondaryAxis></Value></Frame></Frames>
  Cap Top : sm_lib/Body Elements/Cylindrical Solid  CylinderRadius=radius_shock_cyl  CylinderRadiusUnits=m  CylinderLength=cyl_cap_len_shock  CylinderLengthUnits=m  ExportEntireGeometry=off  InertiaType=CalculateFromGeometry  BasedOnType=Density  Density=0  DensityUnits=kg/m^3  Mass=1  MassUnits=kg  CenterOfMass=[0 0 0]  CenterOfMassUnits=m  MomentsOfInertia=[1 1 1]  MomentsOfInertiaUnits=kg*m^2  ProductsOfInertia=[0 0 0]  ProductsOfInertiaUnits=kg*m^2  GraphicType=FromGeometry  MarkerShape=Sphere  MarkerSize=10  GraphicVisPropType=SimpleVisualProperties  GraphicDiffuseColor=clr_shock_cyl  GraphicOpacity=opc_shock_cyl  GraphicSpecularColor=[0.5 0.5 0.5 1.0]  GraphicAmbientColor=[0.15 0.15 0.15 1.0]  GraphicEmissiveColor=[0.0 0.0 0.0 1.0]  GraphicShininess=75  DoExposeReferenceFrame=off  SerializedFrames=<Frames><Frame><Id>Frame2</Id><Value><Name>B</Name><Origin><Source>GeometricFeature</Source><FeatureName>bottom surface</FeatureName></Origin><PrimaryAxis><DefinedDirection>+Z</DefinedDirection><Source>ReferenceFrame</Source><SourceDirection>+Z</SourceDirection><FeatureName></FeatureName></PrimaryAxis><SecondaryAxis><DefinedDirection>+X</DefinedDirection><Source>ReferenceFrame</Source><SourceDirection>+X</SourceDirection><FeatureName></FeatureName></SecondaryAxis></Value></Frame><Frame><Id>Frame1</Id><Value><Name>F</Name><Origin><Source>GeometricFeature</Source><FeatureName>top surface</FeatureName></Origin><PrimaryAxis><DefinedDirection>+Z</DefinedDirection><Source>ReferenceFrame</Source><SourceDirection>+Z</SourceDirection><FeatureName></FeatureName></PrimaryAxis><SecondaryAxis><DefinedDirection>+X</DefinedDirection><Source>ReferenceFrame</Source><SourceDirection>+X</SourceDirection><FeatureName></FeatureName></SecondaryAxis></Value></Frame></Frames>
  Rigid Transform : sm_lib/Frames and Transforms/Rigid Transform  RotationMethod=StandardAxis  FollAlignAxisA=+X  BaseAlignAxisA=+Y  FollAlignAxisB=+Y  BaseAlignAxisB=+Z  RotationStandardAxis=+X  RotationAngle=180  RotationAngleUnits=deg  RotationArbitraryAxis=[0 0 1]  RotationSequenceAxes=FollowerAxes  RotationSequence=XYX  RotationSequenceAngles=[0 0 0]  RotationSequenceAnglesUnits=deg  RotationMatrix=[1 0 0;0 1 0;0 0 1]  Quaternion=[1 0 0 0]  TranslationMethod=None  TranslationCartesianOffset=[0 0 0]  TranslationCartesianOffsetUnits=m  TranslationStandardAxis=+Z  TranslationStandardOffset=0  TranslationStandardOffsetUnits=m  TranslationROffset=0  TranslationROffsetUnits=m  TranslationThetaOffset=0  TranslationThetaOffsetUnits=deg  TranslationZOffset=0  TranslationZOffsetUnits=m
  Wall : sm_lib/Body Elements/Cylindrical Solid  CylinderRadius=radius_shock_cyl  CylinderRadiusUnits=m  CylinderLength=cyl_wall_length  CylinderLengthUnits=m  ExportEntireGeometry=off  InertiaType=CalculateFromGeometry  BasedOnType=Mass  Density=7000/10  DensityUnits=kg/m^3  Mass=shock_cyl_mass  MassUnits=kg  CenterOfMass=[0 0 0]  CenterOfMassUnits=m  MomentsOfInertia=[1 1 1]  MomentsOfInertiaUnits=kg*m^2  ProductsOfInertia=[0 0 0]  ProductsOfInertiaUnits=kg*m^2  GraphicType=FromGeometry  MarkerShape=Sphere  MarkerSize=10  GraphicVisPropType=SimpleVisualProperties  GraphicDiffuseColor=clr_shock_cyl  GraphicOpacity=opc_shock_cyl*0.3  GraphicSpecularColor=[0.5 0.5 0.5 1.0]  GraphicAmbientColor=[0.15 0.15 0.15 1.0]  GraphicEmissiveColor=[0.0 0.0 0.0 1.0]  GraphicShininess=75  DoExposeReferenceFrame=off  SerializedFrames=<Frames><Frame><Id>Frame1</Id><Value><Name>F</Name><Origin><Source>GeometricFeature</Source><FeatureName>top surface</FeatureName></Origin><PrimaryAxis><DefinedDirection>+Z</DefinedDirection><Source>ReferenceFrame</Source><SourceDirection>+Z</SourceDirection><FeatureName></FeatureName></PrimaryAxis><SecondaryAxis><DefinedDirection>+X</DefinedDirection><Source>ReferenceFrame</Source><SourceDirection>+X</SourceDirection><FeatureName></FeatureName></SecondaryAxis></Value></Frame><Frame><Id>Frame2</Id><Value><Name>B</Name><Origin><Source>GeometricFeature</Source><FeatureName>bottom surface</FeatureName></Origin><PrimaryAxis><DefinedDirection>+Z</DefinedDirection><Source>ReferenceFrame</Source><SourceDirection>+Z</SourceDirection><FeatureName></FeatureName></PrimaryAxis><SecondaryAxis><DefinedDirection>+X</DefinedDirection><Source>ReferenceFrame</Source><SourceDirection>+X</SourceDirection><FeatureName></FeatureName></SecondaryAxis></Value></Frame></Frames>
  B : PMIOPort  Side=Left
  connections:
  Wall/RConn1 -- Cap Bottom/LConn1
  Cap Top/LConn1 -- Rigid Transform/RConn1 -- Wall/LConn1
  B/RConn1 -- Rigid Transform/LConn1

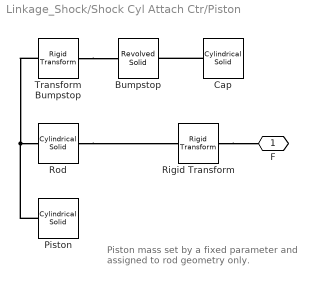
== system Linkage_Shock/Shock Cyl Attach Ctr/Piston ==
  note: Piston mass set by a fixed parameter
      | and assigned to rod geometry only.
  Bumpstop : sm_lib/Body Elements/Revolved Solid  RevolutionCrossSection=bumpstop_xc_rev  RevolutionCrossSectionUnits=m  RevolutionExtent=Full  RevolutionAngle=180  RevolutionAngleUnits=deg  ExportConvexHullGeometry=off  InertiaType=CalculateFromGeometry  BasedOnType=Density  Density=0  DensityUnits=kg/m^3  Mass=1  MassUnits=kg  CenterOfMass=[0 0 0]  CenterOfMassUnits=m  MomentsOfInertia=[1 1 1]  MomentsOfInertiaUnits=kg*m^2  ProductsOfInertia=[0 0 0]  ProductsOfInertiaUnits=kg*m^2  GraphicType=FromGeometry  MarkerShape=Sphere  MarkerSize=10  GraphicVisPropType=SimpleVisualProperties  GraphicDiffuseColor=clr_shock_bumpstop  GraphicOpacity=opc_shock_bumpstop  GraphicSpecularColor=[0.5 0.5 0.5 1.0]  GraphicAmbientColor=[0.15 0.15 0.15 1.0]  GraphicEmissiveColor=[0.0 0.0 0.0 1.0]  GraphicShininess=75  DoExposeReferenceFrame=off  SerializedFrames=<Frames><Frame><Id>Frame1</Id><Value><Name>F</Name><Origin><Source>GeometricFeature</Source><FeatureName>side surface 3</FeatureName></Origin><PrimaryAxis><DefinedDirection>+Z</DefinedDirection><Source>ReferenceFrame</Source><SourceDirection>+Z</SourceDirection><FeatureName></FeatureName></PrimaryAxis><SecondaryAxis><DefinedDirection>+X</DefinedDirection><Source>ReferenceFrame</Source><SourceDirection>+X</SourceDirection><FeatureName></FeatureName></SecondaryAxis></Value></Frame><Frame><Id>Frame2</Id><Value><Name>B</Name><Origin><Source>GeometricFeature</Source><FeatureName>side surface 1</FeatureName></Origin><PrimaryAxis><DefinedDirection>+Z</DefinedDirection><Source>ReferenceFrame</Source><SourceDirection>+Z</SourceDirection><FeatureName></FeatureName></PrimaryAxis><SecondaryAxis><DefinedDirection>+X</DefinedDirection><Source>ReferenceFrame</Source><SourceDirection>+X</SourceDirection><FeatureName></FeatureName></SecondaryAxis></Value></Frame></Frames>
  Cap : sm_lib/Body Elements/Cylindrical Solid  CylinderRadius=radius_shock_cyl  CylinderRadiusUnits=m  CylinderLength=cyl_cap_len_shock  CylinderLengthUnits=m  ExportEntireGeometry=off  InertiaType=CalculateFromGeometry  BasedOnType=Density  Density=0  DensityUnits=kg/m^3  Mass=1  MassUnits=kg  CenterOfMass=[0 0 0]  CenterOfMassUnits=m  MomentsOfInertia=[1 1 1]  MomentsOfInertiaUnits=kg*m^2  ProductsOfInertia=[0 0 0]  ProductsOfInertiaUnits=kg*m^2  GraphicType=FromGeometry  MarkerShape=Sphere  MarkerSize=10  GraphicVisPropType=SimpleVisualProperties  GraphicDiffuseColor=clr_shock_piston  GraphicOpacity=opc_shock_piston  GraphicSpecularColor=[0.5 0.5 0.5 1.0]  GraphicAmbientColor=[0.15 0.15 0.15 1.0]  GraphicEmissiveColor=[0.0 0.0 0.0 1.0]  GraphicShininess=75  DoExposeReferenceFrame=off  SerializedFrames=<Frames><Frame><Id>Frame2</Id><Value><Name>B</Name><Origin><Source>GeometricFeature</Source><FeatureName>bottom surface</FeatureName></Origin><PrimaryAxis><DefinedDirection>+Z</DefinedDirection><Source>ReferenceFrame</Source><SourceDirection>+Z</SourceDirection><FeatureName></FeatureName></PrimaryAxis><SecondaryAxis><DefinedDirection>+X</DefinedDirection><Source>ReferenceFrame</Source><SourceDirection>+X</SourceDirection><FeatureName></FeatureName></SecondaryAxis></Value></Frame></Frames>
  Piston : sm_lib/Body Elements/Cylindrical Solid  CylinderRadius=radius_shock_cyl*0.9  CylinderRadiusUnits=m  CylinderLength=piston_len_shock  CylinderLengthUnits=m  ExportEntireGeometry=off  InertiaType=CalculateFromGeometry  BasedOnType=Density  Density=0  DensityUnits=kg/m^3  Mass=1  MassUnits=kg  CenterOfMass=[0 0 0]  CenterOfMassUnits=m  MomentsOfInertia=[1 1 1]  MomentsOfInertiaUnits=kg*m^2  ProductsOfInertia=[0 0 0]  ProductsOfInertiaUnits=kg*m^2  GraphicType=FromGeometry  MarkerShape=Sphere  MarkerSize=10  GraphicVisPropType=SimpleVisualProperties  GraphicDiffuseColor=clr_shock_piston  GraphicOpacity=opc_shock_piston  GraphicSpecularColor=[0.5 0.5 0.5 1.0]  GraphicAmbientColor=[0.15 0.15 0.15 1.0]  GraphicEmissiveColor=[0.0 0.0 0.0 1.0]  GraphicShininess=75  DoExposeReferenceFrame=off  SerializedFrames=<Frames><Frame><Id>Frame2</Id><Value><Name>B</Name><Origin><Source>GeometricFeature</Source><FeatureName>bottom surface</FeatureName></Origin><PrimaryAxis><DefinedDirection>+Z</DefinedDirection><Source>ReferenceFrame</Source><SourceDirection>+Z</SourceDirection><FeatureName></FeatureName></PrimaryAxis><SecondaryAxis><DefinedDirection>+X</DefinedDirection><Source>ReferenceFrame</Source><SourceDirection>+X</SourceDirection><FeatureName></FeatureName></SecondaryAxis></Value></Frame></Frames>
  Rigid Transform : sm_lib/Frames and Transforms/Rigid Transform  RotationMethod=StandardAxis  FollAlignAxisA=+X  BaseAlignAxisA=+Y  FollAlignAxisB=+Y  BaseAlignAxisB=+Z  RotationStandardAxis=+X  RotationAngle=180  RotationAngleUnits=deg  RotationArbitraryAxis=[0 0 1]  RotationSequenceAxes=FollowerAxes  RotationSequence=XYX  RotationSequenceAngles=[0 0 0]  RotationSequenceAnglesUnits=deg  RotationMatrix=[1 0 0;0 1 0;0 0 1]  Quaternion=[1 0 0 0]  TranslationMethod=None  TranslationCartesianOffset=[0 0 0]  TranslationCartesianOffsetUnits=m  TranslationStandardAxis=+Z  TranslationStandardOffset=0  TranslationStandardOffsetUnits=m  TranslationROffset=0  TranslationROffsetUnits=m  TranslationThetaOffset=0  TranslationThetaOffsetUnits=deg  TranslationZOffset=0  TranslationZOffsetUnits=m
  Rod : sm_lib/Body Elements/Cylindrical Solid  CylinderRadius=radius_shock_cyl*0.2  CylinderRadiusUnits=m  CylinderLength=rod_length  CylinderLengthUnits=m  ExportEntireGeometry=off  InertiaType=CalculateFromGeometry  BasedOnType=Mass  Density=7000  DensityUnits=kg/m^3  Mass=shock_pist_mass  MassUnits=kg  CenterOfMass=[0 0 0]  CenterOfMassUnits=m  MomentsOfInertia=[1 1 1]  MomentsOfInertiaUnits=kg*m^2  ProductsOfInertia=[0 0 0]  ProductsOfInertiaUnits=kg*m^2  GraphicType=FromGeometry  MarkerShape=Sphere  MarkerSize=10  GraphicVisPropType=SimpleVisualProperties  GraphicDiffuseColor=clr_shock_piston  GraphicOpacity=opc_shock_piston  GraphicSpecularColor=[0.5 0.5 0.5 1.0]  GraphicAmbientColor=[0.15 0.15 0.15 1.0]  GraphicEmissiveColor=[0.0 0.0 0.0 1.0]  GraphicShininess=75  DoExposeReferenceFrame=off  SerializedFrames=<Frames><Frame><Id>Frame1</Id><Value><Name>F</Name><Origin><Source>GeometricFeature</Source><FeatureName>top surface</FeatureName></Origin><PrimaryAxis><DefinedDirection>+Z</DefinedDirection><Source>ReferenceFrame</Source><SourceDirection>+Z</SourceDirection><FeatureName></FeatureName></PrimaryAxis><SecondaryAxis><DefinedDirection>+X</DefinedDirection><Source>ReferenceFrame</Source><SourceDirection>+X</SourceDirection><FeatureName></FeatureName></SecondaryAxis></Value></Frame><Frame><Id>Frame2</Id><Value><Name>B</Name><Origin><Source>GeometricFeature</Source><FeatureName>bottom surface</FeatureName></Origin><PrimaryAxis><DefinedDirection>+Z</DefinedDirection><Source>ReferenceFrame</Source><SourceDirection>+Z</SourceDirection><FeatureName></FeatureName></PrimaryAxis><SecondaryAxis><DefinedDirection>+X</DefinedDirection><Source>ReferenceFrame</Source><SourceDirection>+X</SourceDirection><FeatureName></FeatureName></SecondaryAxis></Value></Frame></Frames>
  Transform Bumpstop : sm_lib/Frames and Transforms/Rigid Transform  RotationMethod=None  FollAlignAxisA=+X  BaseAlignAxisA=+Y  FollAlignAxisB=+Y  BaseAlignAxisB=+Z  RotationStandardAxis=+Z  RotationAngle=0.0  RotationAngleUnits=deg  RotationArbitraryAxis=[0 0 1]  RotationSequenceAxes=FollowerAxes  RotationSequence=XYX  RotationSequenceAngles=[0 0 0]  RotationSequenceAnglesUnits=deg  RotationMatrix=[1 0 0; 0 1 0; 0 0 1]  Quaternion=[1 0 0 0]  TranslationMethod=StandardAxis  TranslationCartesianOffset=[0 0 0]  TranslationCartesianOffsetUnits=m  TranslationStandardAxis=+Z  TranslationStandardOffset=piston_len_shock+cyl_cap_len_shock+abs(up_lim_bumpstop)+abs(low_lim_bumpstop)  TranslationStandardOffsetUnits=m  TranslationROffset=0  TranslationROffsetUnits=m  TranslationThetaOffset=0  TranslationThetaOffsetUnits=deg  TranslationZOffset=0  TranslationZOffsetUnits=m
  F : PMIOPort  Side=Right
  connections:
  Transform Bumpstop/RConn1 -- Bumpstop/RConn1
  Cap/LConn1 -- Bumpstop/LConn1
  Rod/LConn1 -- Rigid Transform/LConn1
  Transform Bumpstop/LConn1 -- Piston/LConn1 -- Rod/RConn1
  Rigid Transform/RConn1 -- F/RConn1

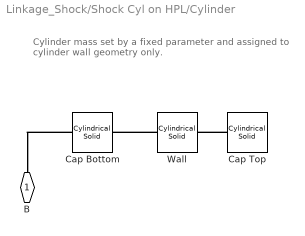
== system Linkage_Shock/Shock Cyl on HPL/Cylinder ==
  note: Cylinder mass set by a fixed parameter
      | and assigned to cylinder wall geometry only.
  Cap Bottom : sm_lib/Body Elements/Cylindrical Solid  CylinderRadius=radius_shock_cyl  CylinderRadiusUnits=m  CylinderLength=cyl_cap_len_shock  CylinderLengthUnits=m  ExportEntireGeometry=off  InertiaType=CalculateFromGeometry  BasedOnType=Density  Density=0  DensityUnits=kg/m^3  Mass=1  MassUnits=kg  CenterOfMass=[0 0 0]  CenterOfMassUnits=m  MomentsOfInertia=[1 1 1]  MomentsOfInertiaUnits=kg*m^2  ProductsOfInertia=[0 0 0]  ProductsOfInertiaUnits=kg*m^2  GraphicType=FromGeometry  MarkerShape=Sphere  MarkerSize=10  GraphicVisPropType=SimpleVisualProperties  GraphicDiffuseColor=clr_shock_cyl  GraphicOpacity=opc_shock_cyl  GraphicSpecularColor=[0.5 0.5 0.5 1.0]  GraphicAmbientColor=[0.15 0.15 0.15 1.0]  GraphicEmissiveColor=[0.0 0.0 0.0 1.0]  GraphicShininess=75  DoExposeReferenceFrame=off  SerializedFrames=<Frames><Frame><Id>Frame1</Id><Value><Name>F</Name><Origin><Source>GeometricFeature</Source><FeatureName>top surface</FeatureName></Origin><PrimaryAxis><DefinedDirection>+Z</DefinedDirection><Source>ReferenceFrame</Source><SourceDirection>+Z</SourceDirection><FeatureName></FeatureName></PrimaryAxis><SecondaryAxis><DefinedDirection>+X</DefinedDirection><Source>ReferenceFrame</Source><SourceDirection>+X</SourceDirection><FeatureName></FeatureName></SecondaryAxis></Value></Frame><Frame><Id>Frame2</Id><Value><Name>B</Name><Origin><Source>GeometricFeature</Source><FeatureName>bottom surface</FeatureName></Origin><PrimaryAxis><DefinedDirection>+Z</DefinedDirection><Source>ReferenceFrame</Source><SourceDirection>+Z</SourceDirection><FeatureName></FeatureName></PrimaryAxis><SecondaryAxis><DefinedDirection>+X</DefinedDirection><Source>ReferenceFrame</Source><SourceDirection>+X</SourceDirection><FeatureName></FeatureName></SecondaryAxis></Value></Frame></Frames>
  Cap Top : sm_lib/Body Elements/Cylindrical Solid  CylinderRadius=radius_shock_cyl  CylinderRadiusUnits=m  CylinderLength=cyl_cap_len_shock  CylinderLengthUnits=m  ExportEntireGeometry=off  InertiaType=CalculateFromGeometry  BasedOnType=Density  Density=0  DensityUnits=kg/m^3  Mass=1  MassUnits=kg  CenterOfMass=[0 0 0]  CenterOfMassUnits=m  MomentsOfInertia=[1 1 1]  MomentsOfInertiaUnits=kg*m^2  ProductsOfInertia=[0 0 0]  ProductsOfInertiaUnits=kg*m^2  GraphicType=FromGeometry  MarkerShape=Sphere  MarkerSize=10  GraphicVisPropType=SimpleVisualProperties  GraphicDiffuseColor=clr_shock_cyl  GraphicOpacity=opc_shock_cyl  GraphicSpecularColor=[0.5 0.5 0.5 1.0]  GraphicAmbientColor=[0.15 0.15 0.15 1.0]  GraphicEmissiveColor=[0.0 0.0 0.0 1.0]  GraphicShininess=75  DoExposeReferenceFrame=off  SerializedFrames=<Frames><Frame><Id>Frame2</Id><Value><Name>B</Name><Origin><Source>GeometricFeature</Source><FeatureName>bottom surface</FeatureName></Origin><PrimaryAxis><DefinedDirection>+Z</DefinedDirection><Source>ReferenceFrame</Source><SourceDirection>+Z</SourceDirection><FeatureName></FeatureName></PrimaryAxis><SecondaryAxis><DefinedDirection>+X</DefinedDirection><Source>ReferenceFrame</Source><SourceDirection>+X</SourceDirection><FeatureName></FeatureName></SecondaryAxis></Value></Frame></Frames>
  Wall : sm_lib/Body Elements/Cylindrical Solid  CylinderRadius=radius_shock_cyl  CylinderRadiusUnits=m  CylinderLength=cyl_wall_length  CylinderLengthUnits=m  ExportEntireGeometry=off  InertiaType=CalculateFromGeometry  BasedOnType=Mass  Density=7000/10  DensityUnits=kg/m^3  Mass=shock_cyl_mass  MassUnits=kg  CenterOfMass=[0 0 0]  CenterOfMassUnits=m  MomentsOfInertia=[1 1 1]  MomentsOfInertiaUnits=kg*m^2  ProductsOfInertia=[0 0 0]  ProductsOfInertiaUnits=kg*m^2  GraphicType=FromGeometry  MarkerShape=Sphere  MarkerSize=10  GraphicVisPropType=SimpleVisualProperties  GraphicDiffuseColor=clr_shock_cyl  GraphicOpacity=opc_shock_cyl*0.3  GraphicSpecularColor=[0.5 0.5 0.5 1.0]  GraphicAmbientColor=[0.15 0.15 0.15 1.0]  GraphicEmissiveColor=[0.0 0.0 0.0 1.0]  GraphicShininess=75  DoExposeReferenceFrame=off  SerializedFrames=<Frames><Frame><Id>Frame1</Id><Value><Name>F</Name><Origin><Source>GeometricFeature</Source><FeatureName>top surface</FeatureName></Origin><PrimaryAxis><DefinedDirection>+Z</DefinedDirection><Source>ReferenceFrame</Source><SourceDirection>+Z</SourceDirection><FeatureName></FeatureName></PrimaryAxis><SecondaryAxis><DefinedDirection>+X</DefinedDirection><Source>ReferenceFrame</Source><SourceDirection>+X</SourceDirection><FeatureName></FeatureName></SecondaryAxis></Value></Frame><Frame><Id>Frame2</Id><Value><Name>B</Name><Origin><Source>GeometricFeature</Source><FeatureName>bottom surface</FeatureName></Origin><PrimaryAxis><DefinedDirection>+Z</DefinedDirection><Source>ReferenceFrame</Source><SourceDirection>+Z</SourceDirection><FeatureName></FeatureName></PrimaryAxis><SecondaryAxis><DefinedDirection>+X</DefinedDirection><Source>ReferenceFrame</Source><SourceDirection>+X</SourceDirection><FeatureName></FeatureName></SecondaryAxis></Value></Frame></Frames>
  B : PMIOPort  Side=Left
  connections:
  Cap Bottom/RConn1 -- B/RConn1
  Cap Top/LConn1 -- Wall/LConn1
  Wall/RConn1 -- Cap Bottom/LConn1
